simulink model "Lat_Dynamics_Simul"  (R2022b)
settings: Solver=FixedStepAuto  StartTime=0.0  StopTime=t_l  FixedStep=0.001  RelTol=1e-3
values from neighbouring files (symbols this model uses):
  Cf_nom = 140000    [Cornering_Stiffness_Tuning.m]    (also in Lat_Dynamics_Simul_initialize.m = 146625; State_Estimator.m = 130000)
  Cr_nom = 160000    [Cornering_Stiffness_Tuning.m]    (also in Lat_Dynamics_Simul_initialize.m = 146400; State_Estimator.m)
  g = 9.81    [Cornering_Stiffness_Tuning.m]    (also in Lat_Dynamics_Simul_initialize.m; State_Estimator.m)
  J = 3495    [Cornering_Stiffness_Tuning.m]    (also in Lat_Dynamics_Simul_initialize.m; State_Estimator.m)
  Lf = 1.15    [Cornering_Stiffness_Tuning.m]    (also in Lat_Dynamics_Simul_initialize.m; State_Estimator.m)
  Lr = 1.49    [Cornering_Stiffness_Tuning.m]    (also in Lat_Dynamics_Simul_initialize.m; State_Estimator.m)
  M = 1523    [Cornering_Stiffness_Tuning.m]    (also in Lat_Dynamics_Simul_initialize.m; State_Estimator.m)
libraries: autolibshared x1
settings Model: Creator=LDW  LastModifiedBy=lego0

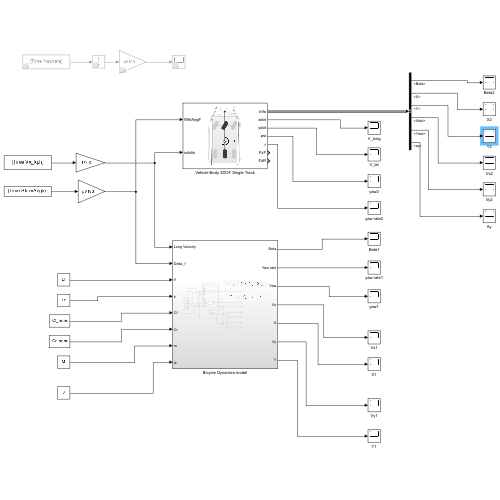
[thumbnail: Simulink's stored preview of the top-level diagram]
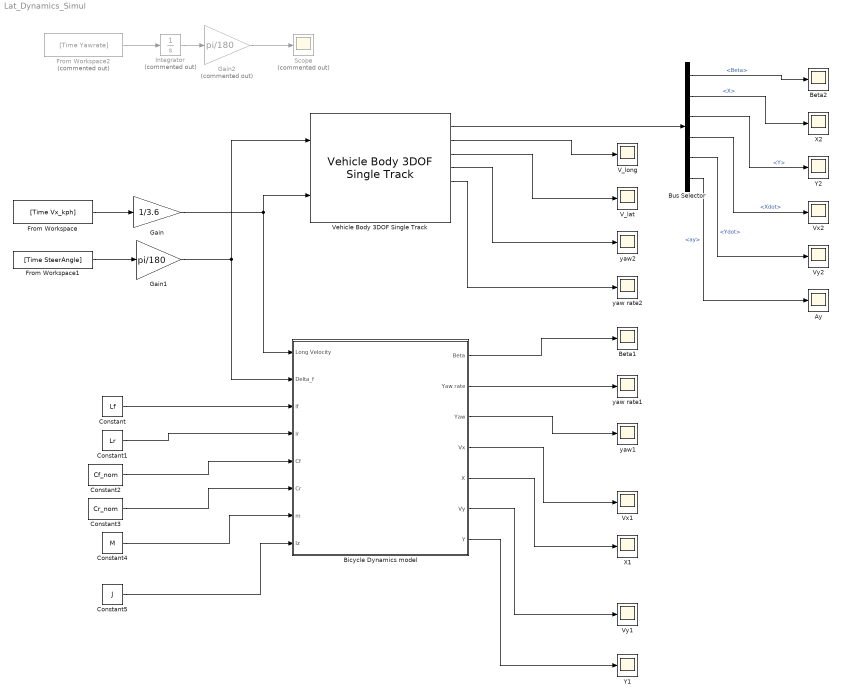
== system Lat_Dynamics_Simul ==
  Ay : Scope
  Beta1 : Scope
  Beta2 : Scope
  Bicycle Dynamics model : Subsystem
  Bus Selector : BusSelector  OutputSignals=BdyFrm.Cg.Ang.Beta,InertFrm.Cg.Disp.X,InertFrm.Cg.Disp.Y,InertFrm.Cg.Vel.Xdot,InertFrm.Cg.Vel.Ydot,BdyFrm.Cg.Acc.ay
  Constant : Constant  Value=Lf
  Constant1 : Constant  Value=Lr
  Constant2 : Constant  Value=Cf_nom
  Constant3 : Constant  Value=Cr_nom
  Constant4 : Constant  Value=M
  Constant5 : Constant  Value=J
  From Workspace : FromWorkspace  VariableName=[Time Vx_kph]
  From Workspace1 : FromWorkspace  VariableName=[Time SteerAngle]
  From Workspace2 : FromWorkspace  Commented=on  VariableName=[Time Yawrate]
  Gain : Gain  Gain=1/3.6
  Gain1 : Gain  Gain=pi/180
  Gain2 : Gain  Commented=on  Gain=pi/180
  Integrator : Integrator  Commented=on
  Scope : Scope  Commented=on
  V_lat : Scope
  V_long : Scope
  Vehicle Body 3DOF Single Track : autolibshared/Vehicle Body 3DOF Single Track  trackMode=Single (bicycle)  inputMode=External longitudinal velocity  frontSteerMode=on  rearSteerMode=off  windMode=off  muMode=off  extFMode=off  extMMode=off  htchFMode=off  htchMMode=off  extXo=off  extpsio=off  extxdoto=off  extro=off  extYo=off  extTamb=off  extydoto=off  aMode=2  NF=2  NR=2  m=M  a=Lf  b=Lr  h=0.35  dh=1  hh=0.2  X_o=0  xdot_o=0  CalphaMode=off  sigmaMode=on  d=0  hl=0  w=[1.4,1.4]  Cy_f=Cf_nom*2  Cy_r=Cr_nom*2  sigma_f=.1  sigma_r=.1  alpha_f_brk=[-.1 .1]  Cy_f_data=[-9e3 9e3]  alpha_r_brk=[-.1 .1]  Cy_r_data=[-9e3 9e3]  Y_o=0  ydot_o=0  Izz=J  psi_o=0  r_o=0  Af=2  Cd=.3  Cl=.1  Cpm=.1  beta_w=[0 0.01:0.01:0.3]  Cs=[0 0.01:0.01:0.3]  Cym=[0 1e-6:0.01:0.3]  Pabs=101325  Tair=273  g=9.81  mu=1  xdot_tol=.01  Fznom=M*g  Fxtire_sat=7e4  Fytire_sat=7e4  longOff=0  latOff=0  vertOff=0  wrapAng=off
  Vx1 : Scope
  Vx2 : Scope
  Vy1 : Scope
  Vy2 : Scope
  X1 : Scope
  X2 : Scope
  Y1 : Scope
  Y2 : Scope
  yaw rate1 : Scope
  yaw rate2 : Scope
  yaw1 : Scope
  yaw2 : Scope
  wires:
  Bus Selector/2 -> X2/1  "<X>"
  Vehicle Body 3DOF Single Track/5 -> yaw rate2/1
  Vehicle Body 3DOF Single Track/4 -> yaw2/1
  Bus Selector/1 -> Beta2/1  "<Beta>"
  Vehicle Body 3DOF Single Track/1 -> Bus Selector/1
  Bus Selector/3 -> Y2/1  "<Y>"
  Vehicle Body 3DOF Single Track/3 -> V_lat/1
  Vehicle Body 3DOF Single Track/2 -> V_long/1
  From Workspace1/1 -> Gain1/1
  Bus Selector/4 -> Vx2/1  "<Xdot>"
  Bus Selector/5 -> Vy2/1  "<Ydot>"
  Constant/1 -> Bicycle Dynamics model/3(lf)
  Constant1/1 -> Bicycle Dynamics model/4(lr)
  Constant2/1 -> Bicycle Dynamics model/5(Cf)
  Constant3/1 -> Bicycle Dynamics model/6(Cr)
  Constant4/1 -> Bicycle Dynamics model/7(m)
  Constant5/1 -> Bicycle Dynamics model/8(Iz)
  Bicycle Dynamics model/1(Beta) -> Beta1/1
  Bicycle Dynamics model/2(Yaw rate) -> yaw rate1/1
  Bicycle Dynamics model/3(Yaw) -> yaw1/1
  Bicycle Dynamics model/4(Vx) -> Vx1/1
  Bicycle Dynamics model/5(X) -> X1/1
  Bicycle Dynamics model/6(Vy) -> Vy1/1
  Bicycle Dynamics model/7(Y) -> Y1/1
  Gain/1 -> Bicycle Dynamics model/1(Long Velocity), Vehicle Body 3DOF Single Track/2
  From Workspace/1 -> Gain/1
  Gain1/1 -> Vehicle Body 3DOF Single Track/1, Bicycle Dynamics model/2(Delta_f)
  Bus Selector/6 -> Ay/1  "<ay>"
  From Workspace2/1 -> Integrator/1
  Integrator/1 -> Gain2/1
  Gain2/1 -> Scope/1

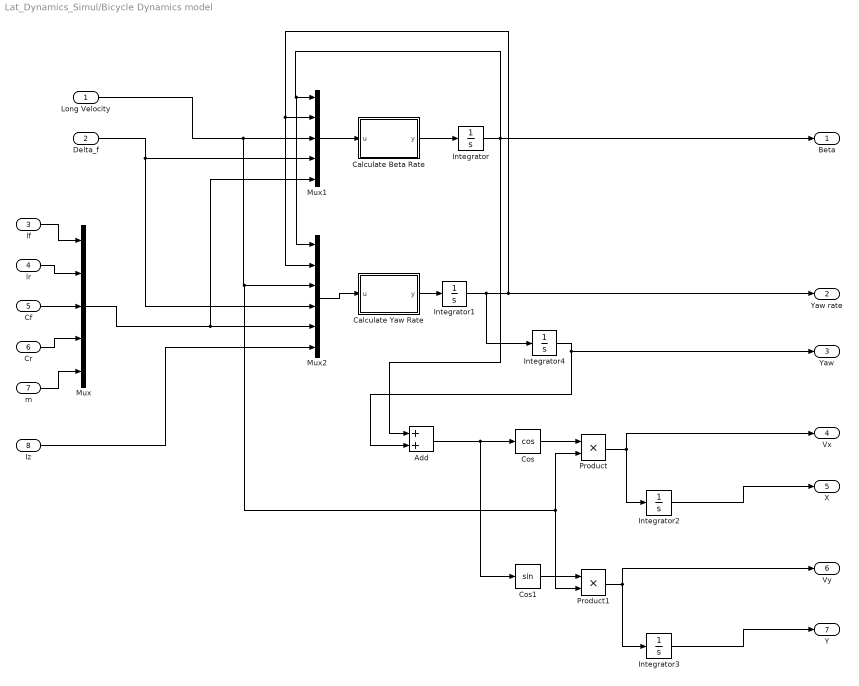
== system Lat_Dynamics_Simul/Bicycle Dynamics model ==
  Long Velocity : Inport
  Delta_f : Inport  Port=2
  lf : Inport  Port=3
  lr : Inport  Port=4
  Cf : Inport  Port=5
  Cr : Inport  Port=6
  m : Inport  Port=7
  Iz : Inport  Port=8
  Add : Sum
  Calculate Beta Rate : MATLAB Function  TreatAsAtomicUnit=on
  Calculate Yaw Rate : MATLAB Function  TreatAsAtomicUnit=on
  Cos : Trigonometry  Operator=cos
  Cos1 : Trigonometry
  Integrator{,1..4} (5 alike) : Integrator
  Mux : Mux  Inputs=5
  Mux1 : Mux  Inputs=5
  Mux2 : Mux  Inputs=6
  Product : Product
  Product1 : Product
  Beta : Outport
  Yaw rate : Outport  Port=2
  Yaw : Outport  Port=3
  Vx : Outport  Port=4
  X : Outport  Port=5
  Vy : Outport  Port=6
  Y : Outport  Port=7
  wires:
  m/1 -> Mux/5
  Cos1/1 -> Product1/1
  Product/1 -> Vx/1, Integrator2/1
  Delta_f/1 -> Mux2/4, Mux1/4
  Add/1 -> Cos1/1, Cos/1
  Mux1/1 -> Calculate Beta Rate/1(u)
  Integrator1/1 -> Integrator4/1, Yaw rate/1, Mux2/2, Mux1/2
  Integrator/1 -> Beta/1, Mux2/1, Mux1/1, Add/1
  Product1/1 -> Vy/1, Integrator3/1
  Mux2/1 -> Calculate Yaw Rate/1(u)
  Calculate Yaw Rate/1(y) -> Integrator1/1
  Integrator4/1 -> Yaw/1, Add/2
  Long Velocity/1 -> Product/2, Product1/2, Mux2/3, Mux1/3
  Mux/1 -> Mux2/5, Mux1/5
  lf/1 -> Mux/1
  Cos/1 -> Product/1
  Calculate Beta Rate/1(y) -> Integrator/1
  Integrator2/1 -> X/1
  lr/1 -> Mux/2
  Cr/1 -> Mux/4
  Cf/1 -> Mux/3
  Iz/1 -> Mux2/6
  Integrator3/1 -> Y/1

== matlab function Lat_Dynamics_Simul/Bicycle Dynamics model/Calculate Beta Rate ==
  data: u input; y output
function y = fcn(u)

beta = u(1);
yaw = u(2);
Vel = u(3);
delta_f = u(4);
lf = u(5);
lr = u(6);
Cf = u(7);
Cr = u(8);
m = u(9);

beta_rate = -(2*Cf+2*Cr)/(m*Vel)*beta + ((2*Cr*lr-2*Cf*lf)/(m*Vel^2)-1)*yaw + 2*Cf/m/Vel*delta_f;


y = beta_rate;

== matlab function Lat_Dynamics_Simul/Bicycle Dynamics model/Calculate Yaw Rate ==
  data: u input; y output
function y = fcn(u)

beta = u(1);
yaw = u(2);
Vel = u(3);
delta_f = u(4);
lf = u(5);
lr = u(6);
Cf = u(7);
Cr = u(8);
m = u(9);
Iz = u(10);

yaw_rate = (-2*lf*Cf+2*lr*Cr)/Iz*beta - (2*Cf*lf^2+2*Cr*lr^2)/(Vel*Iz)*yaw + 2*lf*Cf/Iz*delta_f;


y = yaw_rate;
